simulink library "Turbine_Input_Lib"  (R2025a)
settings: Solver=ode45  StartTime=0.0  StopTime=10.0  RelTol=1e-3  EnableMultiTasking=on
undefined symbols (not defined in the file): sigbuilder_block
libraries: simulink x1, $bdroot x1
Description:
  | Copyright 2009-2025 The MathWorks, Inc. MathWorks, Inc.
settings Model: Creator=smiller  LastModifiedBy=smiller
settings SolverCC: AlgebraicLoopSolver=TrustRegion
settings DataIOCC: LimitDataPoints=on  SaveFormat=Array  SignalLoggingSaveFormat=ModelDataLogs  ReturnWorkspaceOutputs=off
settings OptimizationCC: ReuseModelBlockBuffer=off  ExpressionDepthLimit=2147483647.0  LifeSpan=inf
settings DebuggingCC: UnderspecifiedInitializationDetection=Classic  MergeDetectMultiDrivingBlocksExec=none  SolverPrmCheckMsg=warning  FcnCallInpInsideContextMsg=warning  UnconnectedInputMsg=warning  UnconnectedOutputMsg=warning  UnconnectedLineMsg=warning  AllowSymbolicDim=off  StateNameClashWarn=warning  PregeneratedLibrarySubsystemCodeDiagnostic=none  SFUnexpectedBacktrackingDiag=warning  SFNoUnconditionalDefaultTransitionDiag=warning  SFExecutionAtInitializationDiag=none  ArithmeticOperatorsInVariantConditions=warning
settings HardwareCC: ProdBitPerPointer=32.0  ProdBitPerSizeT=32.0  ProdBitPerPtrDiffT=32.0  ProdLargestAtomicFloat=None  ProdIntDivRoundTo=Undefined  ProdEndianess=Unspecified  ProdWordSize=32.0  ProdHWDeviceType=32-bit Generic
settings ModelReferenceCC: EnableRefExpFcnMdlSchedulingChecks=on  PropagateSignalLabelsOutOfModel=off
settings SFSimCC: SimUseLocalCustomCode=off  CustomCodeUndefinedFunction=UseInterfaceOnly
settings RTWCC: RTWUseLocalCustomCode=off  GPUComputeCapability=3.5  DLArmComputeVersion=19.05
settings CodeAppCC: StateflowObjectComments=on
settings GRTTargetCC: TargetLangStandard=C89/C90 (ANSI)  CombineOutputUpdateFcns=off  GRTInterface=on
settings ConfigComp: CovMetricSettings=dw  CovSaveCumulativeToWorkspaceVar=on  CovSaveSingleToWorkspaceVar=on  CovExternalEMLEnable=off  CovSFcnEnable=off

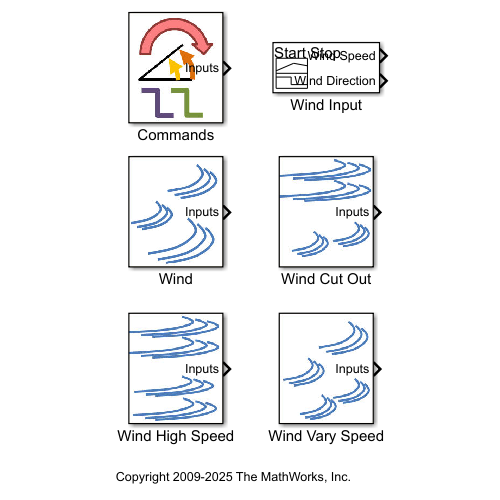
[thumbnail: Simulink's stored preview of the top-level diagram]
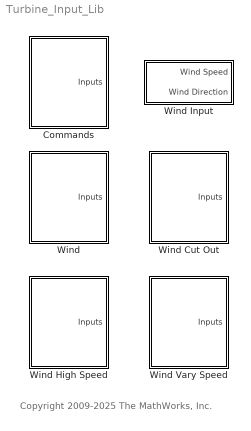
== system Turbine_Input_Lib ==
  note: Copyright 2009-2025 The MathWorks, Inc.
  Commands : Subsystem
      mask Display: image('Turbine_Input_Commands_IMAGE.jpg');
  Wind : Subsystem
      mask Display: image('Turbine_Input_Wind_IMAGE.jpg');
  Wind Cut Out : Subsystem
      mask Display: image('Turbine_Input_Wind_Cut_Out_IMAGE.jpg');
  Wind High Speed : Subsystem
      mask Display: image('Turbine_Input_Wind_High_Speed_IMAGE.jpg');
  Wind Input : Subsystem  Tag=STV Subsys  LoadFcn=sigbuilder_block('load');  StartFcn=sigbuilder_block('start');  StopFcn=sigbuilder_block('stop');  ClipboardFcn=sigbuilder_block('clipboard');  mask(Sigbuilder block){tuvar=[0:10]}
      mask help: Sigbuilder GUI
      mask init:
      | if ~strcmp(get_param(bdroot(gcbh),'SimulationStatus'),'stopped') tuvar = sigbuilder_block('maskInit'); end
      settings: CopyFcn=sigbuilder_block('copy');  DeleteFcn=sigbuilder_block('delete');  ModelCloseFcn=sigbuilder_block('modelClose');  PreSaveFcn=sigbuilder_block('preSave');  PauseFcn=sigbuilder_block('pause')  ContinueFcn=sigbuilder_block('continue')  NameChangeFcn=sigbuilder_block('namechange');  OpenFcn=sigbuilder_block('open',[-3.6 225.6 762 360.6 ]);  CloseFcn=sigbuilder_block('close');
      mask Display: plot(0, 0, 100, 100,[2, 2, 32, 32, 2], [68, 8, 8, 68, 68],[32, 2], [38, 38], [32, 19, 2],[53, 60, 44], [32, 17, 17, 2],[16, 16, 31, 31]);txt = getActiveGroup(gcbh);text(2, 100, txt,'verticalAlignment', 'top');
  Wind Vary Speed : Subsystem
      mask Display: image('Turbine_Input_Wind_Vary_Speed_IMAGE.jpg');

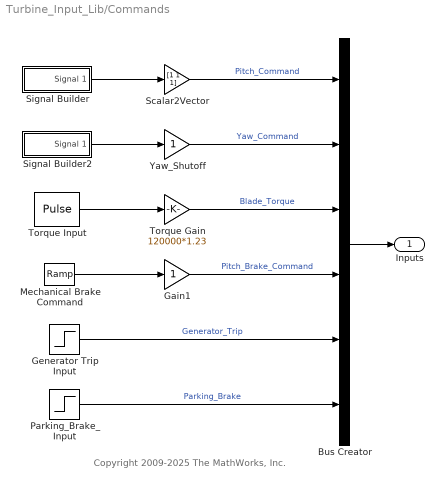
== system Turbine_Input_Lib/Commands ==
  note: Copyright 2009-2025 The MathWorks, Inc.
  Bus Creator : BusCreator  Inputs=6
  Gain1 : Gain
  Generator Trip Input : Step  Time=90  Before=1  SampleTime=0
  Mechanical Brake Command : simulink/Sources/Ramp  slope=1  start=40  InitialOutput=0
  Parking_Brake_Input : Step  Time=5  Before=1  After=0  SampleTime=0
  Scalar2Vector : Gain  Gain=[1 1 1]
  Signal Builder : Subsystem  Tag=STV Subsys  LoadFcn=sigbuilder_block('load');  StartFcn=sigbuilder_block('start');  StopFcn=sigbuilder_block('stop');  ClipboardFcn=sigbuilder_block('clipboard');  mask(Sigbuilder block){tuvar=[0:10]}
      mask help: Sigbuilder GUI
      mask init:
      | if ~strcmp(get_param(bdroot(gcbh),'SimulationStatus'),'stopped') tuvar = sigbuilder_block('maskInit'); end
      settings: CopyFcn=sigbuilder_block('copy');  DeleteFcn=sigbuilder_block('delete');  ModelCloseFcn=sigbuilder_block('modelClose');  PreSaveFcn=sigbuilder_block('preSave');  PauseFcn=sigbuilder_block('pause')  ContinueFcn=sigbuilder_block('continue')  NameChangeFcn=sigbuilder_block('namechange');  OpenFcn=sigbuilder_block('open',[214.5 254.25 550.5 399.75 ]);  CloseFcn=sigbuilder_block('close');
      mask Display: plot(0, 0, 100, 100,[2, 2, 32, 32, 2], [68, 8, 8, 68, 68],[32, 2], [38, 38], [32, 19, 2],[53, 60, 44], [32, 17, 17, 2],[16, 16, 31, 31]);txt = getActiveGroup(gcbh);text(2, 100, txt,'verticalAlignment', 'top');
  Signal Builder2 : Subsystem  Tag=STV Subsys  LoadFcn=sigbuilder_block('load');  StartFcn=sigbuilder_block('start');  StopFcn=sigbuilder_block('stop');  ClipboardFcn=sigbuilder_block('clipboard');  mask(Sigbuilder block){tuvar=[0:10]}
      mask help: Sigbuilder GUI
      mask init:
      | if ~strcmp(get_param(bdroot(gcbh),'SimulationStatus'),'stopped') tuvar = sigbuilder_block('maskInit'); end
      settings: CopyFcn=sigbuilder_block('copy');  DeleteFcn=sigbuilder_block('delete');  ModelCloseFcn=sigbuilder_block('modelClose');  PreSaveFcn=sigbuilder_block('preSave');  PauseFcn=sigbuilder_block('pause')  ContinueFcn=sigbuilder_block('continue')  NameChangeFcn=sigbuilder_block('namechange');  OpenFcn=sigbuilder_block('open',[28.5 161.25 550.5 489 ]);  CloseFcn=sigbuilder_block('close');
      mask Display: plot(0, 0, 100, 100,[2, 2, 32, 32, 2], [68, 8, 8, 68, 68],[32, 2], [38, 38], [32, 19, 2],[53, 60, 44], [32, 17, 17, 2],[16, 16, 31, 31]);txt = getActiveGroup(gcbh);text(2, 100, txt,'verticalAlignment', 'top');
  Torque Gain : Gain  Gain=120000*1.23
  Torque Input : DiscretePulseGenerator  PulseType=Time based  Amplitude=10  Period=100  PulseWidth=10
  Yaw_Shutoff : Gain
  Inputs : Outport  VectorParamsAs1DForOutWhenUnconnected=off
  wires:
  Parking_Brake_Input/1 -> Bus Creator/6  "Parking_Brake"
  Gain1/1 -> Bus Creator/4  "Pitch_Brake_Command"
  Generator Trip Input/1 -> Bus Creator/5  "Generator_Trip"
  Mechanical Brake Command/1 -> Gain1/1
  Torque Gain/1 -> Bus Creator/3  "Blade_Torque"
  Yaw_Shutoff/1 -> Bus Creator/2  "Yaw_Command"
  Scalar2Vector/1 -> Bus Creator/1  "Pitch_Command"
  Torque Input/1 -> Torque Gain/1
  Signal Builder/1(Signal 1) -> Scalar2Vector/1
  Signal Builder2/1(Signal 1) -> Yaw_Shutoff/1
  Bus Creator/1 -> Inputs/1

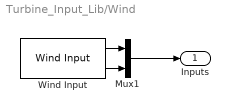
== system Turbine_Input_Lib/Wind ==
  Mux1 : Mux  Inputs=2
  Wind Input : $bdroot/Wind Input  Tag=STV Subsys  tuvar=[0:10]
  Inputs : Outport  VectorParamsAs1DForOutWhenUnconnected=off
  wires:
  Mux1/1 -> Inputs/1
  Wind Input/1 -> Mux1/1
  Wind Input/2 -> Mux1/2

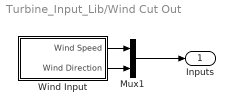
== system Turbine_Input_Lib/Wind Cut Out ==
  Mux1 : Mux  Inputs=2
  Wind Input : Subsystem  Tag=STV Subsys  AncestorBlock=Turbine_Input_Lib/Wind Input  LoadFcn=sigbuilder_block('load');  StartFcn=sigbuilder_block('start');  StopFcn=sigbuilder_block('stop');  ClipboardFcn=sigbuilder_block('clipboard');  mask(Sigbuilder block){}
      mask help: Sigbuilder GUI
      mask init:
      | if ~strcmp(get_param(bdroot(gcbh),'SimulationStatus'),'stopped') tuvar = sigbuilder_block('maskInit'); end
      settings: LibrarySourceBlock=Turbine_Input_Lib/Wind Input  CopyFcn=sigbuilder_block('copy');  DeleteFcn=sigbuilder_block('delete');  ModelCloseFcn=sigbuilder_block('modelClose');  PreSaveFcn=sigbuilder_block('preSave');  PauseFcn=sigbuilder_block('pause')  ContinueFcn=sigbuilder_block('continue')  NameChangeFcn=sigbuilder_block('namechange');  OpenFcn=sigbuilder_block('open',[-3.6 225.6 762 360.6 ]);  CloseFcn=sigbuilder_block('close');
      mask Display: plot(0, 0, 100, 100,[2, 2, 32, 32, 2], [68, 8, 8, 68, 68],[32, 2], [38, 38], [32, 19, 2],[53, 60, 44], [32, 17, 17, 2],[16, 16, 31, 31]);txt = getActiveGroup(gcbh);text(2, 100, txt,'verticalAlignment', 'top');
  Inputs : Outport  VectorParamsAs1DForOutWhenUnconnected=off
  wires:
  Mux1/1 -> Inputs/1
  Wind Input/1(Wind Speed) -> Mux1/1
  Wind Input/2(Wind Direction) -> Mux1/2

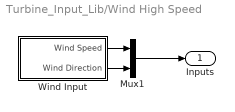
== system Turbine_Input_Lib/Wind High Speed ==
  Mux1 : Mux  Inputs=2
  Wind Input : Subsystem  Tag=STV Subsys  AncestorBlock=Turbine_Input_Lib/Wind Input  LoadFcn=sigbuilder_block('load');  StartFcn=sigbuilder_block('start');  StopFcn=sigbuilder_block('stop');  ClipboardFcn=sigbuilder_block('clipboard');  mask(Sigbuilder block){}
      mask help: Sigbuilder GUI
      mask init:
      | if ~strcmp(get_param(bdroot(gcbh),'SimulationStatus'),'stopped') tuvar = sigbuilder_block('maskInit'); end
      settings: LibrarySourceBlock=Turbine_Input_Lib/Wind Input  CopyFcn=sigbuilder_block('copy');  DeleteFcn=sigbuilder_block('delete');  ModelCloseFcn=sigbuilder_block('modelClose');  PreSaveFcn=sigbuilder_block('preSave');  PauseFcn=sigbuilder_block('pause')  ContinueFcn=sigbuilder_block('continue')  NameChangeFcn=sigbuilder_block('namechange');  OpenFcn=sigbuilder_block('open',[-3.6 225.6 762 360.6 ]);  CloseFcn=sigbuilder_block('close');
      mask Display: plot(0, 0, 100, 100,[2, 2, 32, 32, 2], [68, 8, 8, 68, 68],[32, 2], [38, 38], [32, 19, 2],[53, 60, 44], [32, 17, 17, 2],[16, 16, 31, 31]);txt = getActiveGroup(gcbh);text(2, 100, txt,'verticalAlignment', 'top');
  Inputs : Outport  VectorParamsAs1DForOutWhenUnconnected=off
  wires:
  Wind Input/2(Wind Direction) -> Mux1/2
  Wind Input/1(Wind Speed) -> Mux1/1
  Mux1/1 -> Inputs/1

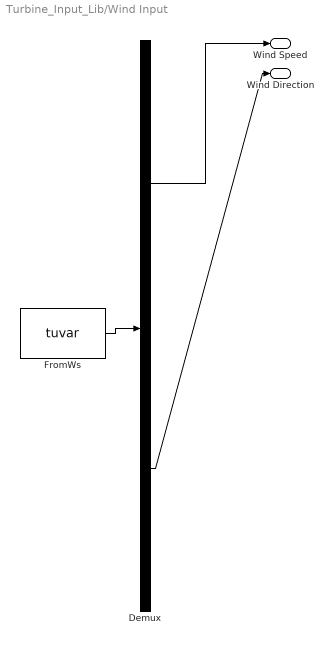
== system Turbine_Input_Lib/Wind Input ==
  Demux : Demux  Tag=STV Demux  Outputs=2
      settings: DisplayOption=none
  FromWs : FromWorkspace  Tag=STV FromWs  VariableName=tuvar
      SigBuilderData=|
      | common.afterFinalStr = 'Extrapolate'
      | common.sampleTime = 0
      | dataSet(1).timeRange = [0 130]
      | dataSet(1).name = 'Constant Wind No Yaw'
      | dataSet(2).timeRange = [0 130]
      | dataSet(2).name = 'Constant Wind'
      | dataSet(3).timeRange = [0 130]
      | dataSet(3).name = 'High WS No Yaw'
      | dataSet(4).timeRange = [0 60]
      | dataSet(4).name = 'High Wind Speed'
      | dataSet(5).timeRange = [0 130]
      | dataSet(5).name = 'Cut Out'
      | dataSet(6).timeRange = [0 130]
      | dataSet(6).name = 'Start Stop'
      | dataSet(7).timeRange = [0 130]
      | dataSet(7).name = 'Start Stop No Yaw'
      | sbobj.Groups(1).Name = 'Constant Wind No Yaw'
      | sbobj.Groups(1).Signals(1).Name = 'Wind Speed'
      | sbobj.Groups(1).Signals(1).XData = [0 10 130]
      | sbobj.Groups(1).Signals(1).YData = [10 10 10]
      | sbobj.Groups(1).Signals(2).Name = 'Wind Direction'
      | sbobj.Groups(1).Signals(2).XData = [0 1 11 21 31 130]
      | sbobj.Groups(1).Signals(2).YData = [0 0 0 0 0 0]
      | sbobj.Groups(1).TimeRange = [0 130]
      | sbobj.Groups(2).Name = 'Constant Wind'
      | sbobj.Groups(2).Signals(1).Name = 'Wind Speed'
      | sbobj.Groups(2).Signals(1).XData = [0 10 130]
      | sbobj.Groups(2).Signals(1).YData = [10 10 10]
      | sbobj.Groups(2).Signals(2).Name = 'Wind Direction'
      | sbobj.Groups(2).Signals(2).XData = [0 1 1 11 11 21 21 31 31 130]
      | sbobj.Groups(2).Signals(2).YData = [0 0 4 4 0 0 -4 -4 0 0]
      | sbobj.Groups(2).TimeRange = [0 130]
      | sbobj.Groups(3).Name = 'High WS No Yaw'
      | sbobj.Groups(3).Signals(1).Name = 'Wind Speed'
      | sbobj.Groups(3).Signals(1).XData = [0 10 10 25.1 28 91.8 100 130]
      | sbobj.Groups(3).Signals(1).YData = [10 10 9.9 9.9 5 5 8 10]
      | sbobj.Groups(3).Signals(2).Name = 'Wind Direction'
      | sbobj.Groups(3).Signals(2).XData = [0 1 11 21 21 31 31 130]
      | sbobj.Groups(3).Signals(2).YData = [0 0 0 0 0 0 0 0]
      | sbobj.Groups(3).TimeRange = [0 130]
      | sbobj.Groups(4).Name = 'High Wind Speed'
      | sbobj.Groups(4).Signals(1).Name = 'Wind Speed'
      | sbobj.Groups(4).Signals(1).XData = [0 10 60]
      | sbobj.Groups(4).Signals(1).YData = [10 9.9 25]
      | sbobj.Groups(4).Signals(2).Name = 'Wind Direction'
      | sbobj.Groups(4).Signals(2).XData = [0 1 11 21 31 60]
      | sbobj.Groups(4).Signals(2).YData = [0 0 4 0 -2.1 0]
      | sbobj.Groups(4).TimeRange = [0 60]
      | sbobj.Groups(5).Name = 'Cut Out'
      | sbobj.Groups(5).Signals(1).Name = 'Wind Speed'
      | sbobj.Groups(5).Signals(1).XData = [0 5 25.1 28 60 75 121.8 130]
      | sbobj.Groups(5).Signals(1).YData = [10 10 8.7 7.85 9.65 2 2 2]
      | sbobj.Groups(5).Signals(2).Name = 'Wind Direction'
      | sbobj.Groups(5).Signals(2).XData = [0 1 1 11 11 21 21 31 31 130]
      | sbobj.Groups(5).Signals(2).YData = [0 0 4 4 0 0 -4 -4 0 0]
      | sbobj.Groups(5).TimeRange = [0 130]
      | sbobj.Groups(6).Name = 'Start Stop'
      | sbobj.Groups(6).Signals(1).Name = 'Wind Speed'
      | sbobj.Groups(6).Signals(1).XData = [0 5 25 28 55 75 80 130]
      | sbobj.Groups(6).Signals(1).YData = [2 2 13 10 15 2 2 2]
      | sbobj.Groups(6).Signals(2).Name = 'Wind Direction'
      | sbobj.Groups(6).Signals(2).XData = [0 1 11 21 31 36.6 54.8 75 130]
      | sbobj.Groups(6).Signals(2).YData = [0 0 2.9 0.5 0.5 1.57171717172 -4 -4 -4]
      | sbobj.Groups(6).TimeRange = [0 130]
      | sbobj.Groups(7).Name = 'Start Stop No Yaw'
      | sbobj.Groups(7).Signals(1).Name = 'Wind Speed'
      | sbobj.Groups(7).Signals(1).XData = [0 5 25 28 55 75 80 130]
      | sbobj.Groups(7).Signals(1).YData = [2 2 13 10 15 2 2 2]
      | sbobj.Groups(7).Signals(2).Name = 'Wind Direction'
      | sbobj.Groups(7).Signals(2).XData = [0 130]
      | sbobj.Groups(7).Signals(2).YData = [0 0]
      | sbobj.Groups(7).TimeRange = [0 130]
  Wind Speed : Outport  Tag=STV Outport  VectorParamsAs1DForOutWhenUnconnected=off
  Wind Direction : Outport  Tag=STV Outport  Port=2  VectorParamsAs1DForOutWhenUnconnected=off
  wires:
  Demux/2 -> Wind Direction/1
  Demux/1 -> Wind Speed/1
  FromWs/1 -> Demux/1

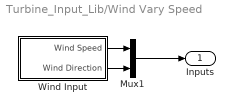
== system Turbine_Input_Lib/Wind Vary Speed ==
  Mux1 : Mux  Inputs=2
  Wind Input : Subsystem  Tag=STV Subsys  AncestorBlock=Turbine_Input_Lib/Wind Input  LoadFcn=sigbuilder_block('load');  StartFcn=sigbuilder_block('start');  StopFcn=sigbuilder_block('stop');  ClipboardFcn=sigbuilder_block('clipboard');  mask(Sigbuilder block){}
      mask help: Sigbuilder GUI
      mask init:
      | if ~strcmp(get_param(bdroot(gcbh),'SimulationStatus'),'stopped') tuvar = sigbuilder_block('maskInit'); end
      settings: LibrarySourceBlock=Turbine_Input_Lib/Wind Input  CopyFcn=sigbuilder_block('copy');  DeleteFcn=sigbuilder_block('delete');  ModelCloseFcn=sigbuilder_block('modelClose');  PreSaveFcn=sigbuilder_block('preSave');  PauseFcn=sigbuilder_block('pause')  ContinueFcn=sigbuilder_block('continue')  NameChangeFcn=sigbuilder_block('namechange');  OpenFcn=sigbuilder_block('open',[-3.6 225.6 762 360.6 ]);  CloseFcn=sigbuilder_block('close');
      mask Display: plot(0, 0, 100, 100,[2, 2, 32, 32, 2], [68, 8, 8, 68, 68],[32, 2], [38, 38], [32, 19, 2],[53, 60, 44], [32, 17, 17, 2],[16, 16, 31, 31]);txt = getActiveGroup(gcbh);text(2, 100, txt,'verticalAlignment', 'top');
  Inputs : Outport  VectorParamsAs1DForOutWhenUnconnected=off
  wires:
  Wind Input/2(Wind Direction) -> Mux1/2
  Wind Input/1(Wind Speed) -> Mux1/1
  Mux1/1 -> Inputs/1

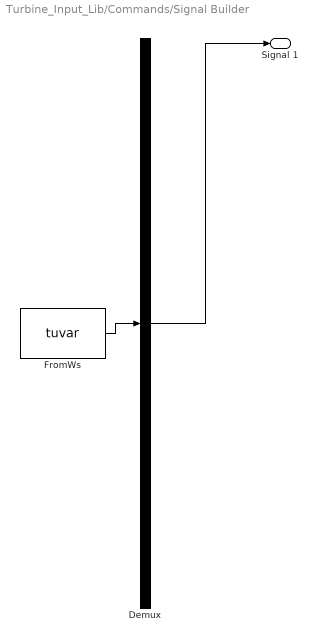
== system Turbine_Input_Lib/Commands/Signal Builder ==
  Demux : Demux  Tag=STV Demux  Outputs=1
      settings: DisplayOption=none
  FromWs : FromWorkspace  Tag=STV FromWs  VariableName=tuvar
      SigBuilderData=|
      | common.afterFinalStr = 'Extrapolate'
      | common.sampleTime = 0
      | dataSet(1).timeRange = [0 50]
      | dataSet(1).name = 'Pos_Test'
      | dataSet(2).timeRange = [0 50]
      | dataSet(2).name = 'Pos_Neg_Test'
      | dataSet(3).timeRange = [0 50]
      | dataSet(3).name = 'Step_Test'
      | sbobj.Groups(1).Name = 'Pos_Test'
      | sbobj.Groups(1).Signals.Name = 'Signal 1'
      | sbobj.Groups(1).Signals.XData = [0 5 5 7.5 7.5 25.1 25.1 28 28 50]
      | sbobj.Groups(1).Signals.YData = [0 0 20 20 0 0 20 20 0 0]
      | sbobj.Groups(1).TimeRange = [0 50]
      | sbobj.Groups(2).Name = 'Pos_Neg_Test'
      | sbobj.Groups(2).Signals.Name = 'Signal 1'
      | sbobj.Groups(2).Signals.XData = [0 3 3 5.5 5.5 8 8 10.5 10.5 50]
      | sbobj.Groups(2).Signals.YData = [0 0 20 20 0 0 -20 -20 0 0]
      | sbobj.Groups(2).TimeRange = [0 50]
      | sbobj.Groups(3).Name = 'Step_Test'
      | sbobj.Groups(3).Signals.Name = 'Signal 1'
      | sbobj.Groups(3).Signals.XData = [0 1 1 7.5 25.1 30 30 50]
      | sbobj.Groups(3).Signals.YData = [0 0 20 20 20 20 0 0]
      | sbobj.Groups(3).TimeRange = [0 50]
  Signal 1 : Outport  Tag=STV Outport  VectorParamsAs1DForOutWhenUnconnected=off
  wires:
  FromWs/1 -> Demux/1
  Demux/1 -> Signal 1/1

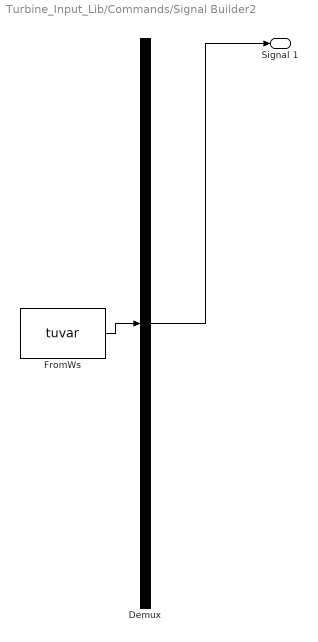
== system Turbine_Input_Lib/Commands/Signal Builder2 ==
  Demux : Demux  Tag=STV Demux  Outputs=1
      settings: DisplayOption=none
  FromWs : FromWorkspace  Tag=STV FromWs  VariableName=tuvar
      SigBuilderData=|
      | common.afterFinalStr = 'Extrapolate'
      | common.sampleTime = 0
      | dataSet(1).timeRange = [0 50]
      | dataSet(1).name = 'Pos_Neg_Test'
      | dataSet(2).timeRange = [0 50]
      | dataSet(2).name = 'Step_Test'
      | dataSet(3).timeRange = [0 50]
      | dataSet(3).name = 'Ramp_Test'
      | sbobj.Groups(1).Name = 'Pos_Neg_Test'
      | sbobj.Groups(1).Signals.Name = 'Signal 1'
      | sbobj.Groups(1).Signals.XData = [0 1 1 11 11 21 21 31 31 50]
      | sbobj.Groups(1).Signals.YData = [0 0 4 4 0 0 -4 -4 0 0]
      | sbobj.Groups(2).Name = 'Step_Test'
      | sbobj.Groups(2).Signals.Name = 'Signal 1'
      | sbobj.Groups(2).Signals.XData = [0 1 1 11 21 31 31 50]
      | sbobj.Groups(2).Signals.YData = [0 0 4 4 4 4 0 0]
      | sbobj.Groups(3).Name = 'Ramp_Test'
      | sbobj.Groups(3).Signals.Name = 'Signal 1'
      | sbobj.Groups(3).Signals.XData = [0 1 1 11 21 31 39.1 50]
      | sbobj.Groups(3).Signals.YData = [0 0 2.46 4 2.32 3.18 1.16 0]
  Signal 1 : Outport  Tag=STV Outport  VectorParamsAs1DForOutWhenUnconnected=off
  wires:
  FromWs/1 -> Demux/1
  Demux/1 -> Signal 1/1

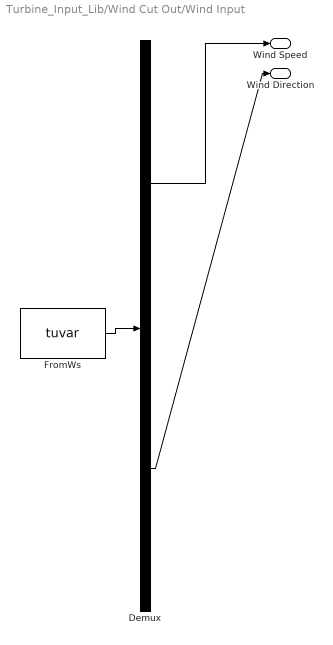
== system Turbine_Input_Lib/Wind Cut Out/Wind Input ==
  Demux : Demux  Tag=STV Demux  Outputs=2
      settings: DisplayOption=none
  FromWs : FromWorkspace  Tag=STV FromWs  VariableName=tuvar
      SigBuilderData=|
      | common.afterFinalStr = 'Extrapolate'
      | common.sampleTime = 0
      | dataSet(1).timeRange = [0 130]
      | dataSet(1).name = 'Constant Wind No Yaw'
      | dataSet(2).timeRange = [0 130]
      | dataSet(2).name = 'Constant Wind'
      | dataSet(3).timeRange = [0 60]
      | dataSet(3).name = 'High Wind Speed'
      | dataSet(4).timeRange = [0 130]
      | dataSet(4).name = 'Cut Out'
      | dataSet(5).timeRange = [0 130]
      | dataSet(5).name = 'Start Stop'
      | dataSet(6).timeRange = [0 130]
      | dataSet(6).name = 'Start Stop No Yaw'
      | dataSet(7).timeRange = [0 130]
      | dataSet(7).name = 'Varying Wind'
      | sbobj.Groups(1).Name = 'Constant Wind No Yaw'
      | sbobj.Groups(1).Signals(1).Name = 'Wind Speed'
      | sbobj.Groups(1).Signals(1).XData = [0 10 130]
      | sbobj.Groups(1).Signals(1).YData = [10 10 10]
      | sbobj.Groups(1).Signals(2).Name = 'Wind Direction'
      | sbobj.Groups(1).Signals(2).XData = [0 1 11 21 31 130]
      | sbobj.Groups(1).Signals(2).YData = [0 0 0 0 0 0]
      | sbobj.Groups(1).TimeRange = [0 130]
      | sbobj.Groups(2).Name = 'Constant Wind'
      | sbobj.Groups(2).Signals(1).Name = 'Wind Speed'
      | sbobj.Groups(2).Signals(1).XData = [0 10 130]
      | sbobj.Groups(2).Signals(1).YData = [10 10 10]
      | sbobj.Groups(2).Signals(2).Name = 'Wind Direction'
      | sbobj.Groups(2).Signals(2).XData = [0 1 1 11 11 21 21 31 31 130]
      | sbobj.Groups(2).Signals(2).YData = [0 0 4 4 0 0 -4 -4 0 0]
      | sbobj.Groups(2).TimeRange = [0 130]
      | sbobj.Groups(3).Name = 'High Wind Speed'
      | sbobj.Groups(3).Signals(1).Name = 'Wind Speed'
      | sbobj.Groups(3).Signals(1).XData = [0 10 60]
      | sbobj.Groups(3).Signals(1).YData = [10 9.9 25]
      | sbobj.Groups(3).Signals(2).Name = 'Wind Direction'
      | sbobj.Groups(3).Signals(2).XData = [0 1 11 21 31 60]
      | sbobj.Groups(3).Signals(2).YData = [0 0 4 0 -2.1 0]
      | sbobj.Groups(3).TimeRange = [0 60]
      | sbobj.Groups(4).Name = 'Cut Out'
      | sbobj.Groups(4).Signals(1).Name = 'Wind Speed'
      | sbobj.Groups(4).Signals(1).XData = [0 5 25.1 28 60 75 121.8 130]
      | sbobj.Groups(4).Signals(1).YData = [10 10 8.7 7.85 9.65 2 2 2]
      | sbobj.Groups(4).Signals(2).Name = 'Wind Direction'
      | sbobj.Groups(4).Signals(2).XData = [0 1 1 11 11 21 21 31 31 130]
      | sbobj.Groups(4).Signals(2).YData = [0 0 4 4 0 0 -4 -4 0 0]
      | sbobj.Groups(4).TimeRange = [0 130]
      | sbobj.Groups(5).Name = 'Start Stop'
      | sbobj.Groups(5).Signals(1).Name = 'Wind Speed'
      | sbobj.Groups(5).Signals(1).XData = [0 5 25 28 55 75 80 130]
      | sbobj.Groups(5).Signals(1).YData = [2 2 13 10 15 2 2 2]
      | sbobj.Groups(5).Signals(2).Name = 'Wind Direction'
      | sbobj.Groups(5).Signals(2).XData = [0 1 11 21 31 36.6 54.8 75 130]
      | sbobj.Groups(5).Signals(2).YData = [0 0 2.9 0.5 0.5 1.57171717172 -4 -4 -4]
      | sbobj.Groups(5).TimeRange = [0 130]
      | sbobj.Groups(6).Name = 'Start Stop No Yaw'
      | sbobj.Groups(6).Signals(1).Name = 'Wind Speed'
      | sbobj.Groups(6).Signals(1).XData = [0 5 25 28 55 75 80 130]
      | sbobj.Groups(6).Signals(1).YData = [2 2 13 10 15 2 2 2]
      | sbobj.Groups(6).Signals(2).Name = 'Wind Direction'
      | sbobj.Groups(6).Signals(2).XData = [0 130]
      | sbobj.Groups(6).Signals(2).YData = [0 0]
      | sbobj.Groups(6).TimeRange = [0 130]
      | sbobj.Groups(7).Name = 'Varying Wind'
      | sbobj.Groups(7).Signals(1).Name = 'Wind Speed'
      | sbobj.Groups(7).Signals(1).XData = [0 5 25 28 45 60.2 75 78.2 80 130]
      | sbobj.Groups(7).Signals(1).YData = [2 2 13 10 14.4 10.6 13.9 8 8 2]
      | sbobj.Groups(7).Signals(2).Name = 'Wind Direction'
      | sbobj.Groups(7).Signals(2).XData = [0 1 11 21 31 36.6 54.8 75 130]
      | sbobj.Groups(7).Signals(2).YData = [0 0 2.9 0.5 0.5 1.57171717172 -4 -4 -4]
      | sbobj.Groups(7).TimeRange = [0 130]
  Wind Speed : Outport  Tag=STV Outport  VectorParamsAs1DForOutWhenUnconnected=off
  Wind Direction : Outport  Tag=STV Outport  Port=2  VectorParamsAs1DForOutWhenUnconnected=off
  wires:
  Demux/2 -> Wind Direction/1
  Demux/1 -> Wind Speed/1
  FromWs/1 -> Demux/1

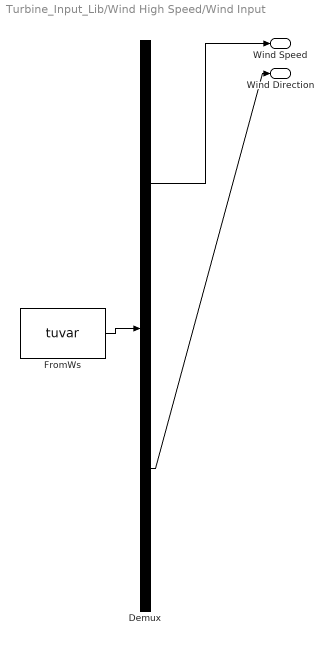
== system Turbine_Input_Lib/Wind High Speed/Wind Input ==
  Demux : Demux  Tag=STV Demux  Outputs=2
      settings: DisplayOption=none
  FromWs : FromWorkspace  Tag=STV FromWs  VariableName=tuvar
      SigBuilderData=|
      | common.afterFinalStr = 'Extrapolate'
      | common.sampleTime = 0
      | dataSet(1).timeRange = [0 130]
      | dataSet(1).name = 'Constant Wind No Yaw'
      | dataSet(2).timeRange = [0 130]
      | dataSet(2).name = 'Constant Wind'
      | dataSet(3).timeRange = [0 60]
      | dataSet(3).name = 'High Wind Speed'
      | dataSet(4).timeRange = [0 130]
      | dataSet(4).name = 'Cut Out'
      | dataSet(5).timeRange = [0 130]
      | dataSet(5).name = 'Start Stop'
      | dataSet(6).timeRange = [0 130]
      | dataSet(6).name = 'Start Stop No Yaw'
      | dataSet(7).timeRange = [0 130]
      | dataSet(7).name = 'Varying Wind'
      | sbobj.Groups(1).Name = 'Constant Wind No Yaw'
      | sbobj.Groups(1).Signals(1).Name = 'Wind Speed'
      | sbobj.Groups(1).Signals(1).XData = [0 10 130]
      | sbobj.Groups(1).Signals(1).YData = [10 10 10]
      | sbobj.Groups(1).Signals(2).Name = 'Wind Direction'
      | sbobj.Groups(1).Signals(2).XData = [0 1 11 21 31 130]
      | sbobj.Groups(1).Signals(2).YData = [0 0 0 0 0 0]
      | sbobj.Groups(1).TimeRange = [0 130]
      | sbobj.Groups(2).Name = 'Constant Wind'
      | sbobj.Groups(2).Signals(1).Name = 'Wind Speed'
      | sbobj.Groups(2).Signals(1).XData = [0 10 130]
      | sbobj.Groups(2).Signals(1).YData = [10 10 10]
      | sbobj.Groups(2).Signals(2).Name = 'Wind Direction'
      | sbobj.Groups(2).Signals(2).XData = [0 1 1 11 11 21 21 31 31 130]
      | sbobj.Groups(2).Signals(2).YData = [0 0 4 4 0 0 -4 -4 0 0]
      | sbobj.Groups(2).TimeRange = [0 130]
      | sbobj.Groups(3).Name = 'High Wind Speed'
      | sbobj.Groups(3).Signals(1).Name = 'Wind Speed'
      | sbobj.Groups(3).Signals(1).XData = [0 10 60]
      | sbobj.Groups(3).Signals(1).YData = [10 9.9 25]
      | sbobj.Groups(3).Signals(2).Name = 'Wind Direction'
      | sbobj.Groups(3).Signals(2).XData = [0 1 11 21 31 60]
      | sbobj.Groups(3).Signals(2).YData = [0 0 4 0 -2.1 0]
      | sbobj.Groups(3).TimeRange = [0 60]
      | sbobj.Groups(4).Name = 'Cut Out'
      | sbobj.Groups(4).Signals(1).Name = 'Wind Speed'
      | sbobj.Groups(4).Signals(1).XData = [0 5 25.1 28 60 75 121.8 130]
      | sbobj.Groups(4).Signals(1).YData = [10 10 8.7 7.85 9.65 2 2 2]
      | sbobj.Groups(4).Signals(2).Name = 'Wind Direction'
      | sbobj.Groups(4).Signals(2).XData = [0 1 1 11 11 21 21 31 31 130]
      | sbobj.Groups(4).Signals(2).YData = [0 0 4 4 0 0 -4 -4 0 0]
      | sbobj.Groups(4).TimeRange = [0 130]
      | sbobj.Groups(5).Name = 'Start Stop'
      | sbobj.Groups(5).Signals(1).Name = 'Wind Speed'
      | sbobj.Groups(5).Signals(1).XData = [0 5 25 28 55 75 80 130]
      | sbobj.Groups(5).Signals(1).YData = [2 2 13 10 15 2 2 2]
      | sbobj.Groups(5).Signals(2).Name = 'Wind Direction'
      | sbobj.Groups(5).Signals(2).XData = [0 1 11 21 31 36.6 54.8 75 130]
      | sbobj.Groups(5).Signals(2).YData = [0 0 2.9 0.5 0.5 1.57171717172 -4 -4 -4]
      | sbobj.Groups(5).TimeRange = [0 130]
      | sbobj.Groups(6).Name = 'Start Stop No Yaw'
      | sbobj.Groups(6).Signals(1).Name = 'Wind Speed'
      | sbobj.Groups(6).Signals(1).XData = [0 5 25 28 55 75 80 130]
      | sbobj.Groups(6).Signals(1).YData = [2 2 13 10 15 2 2 2]
      | sbobj.Groups(6).Signals(2).Name = 'Wind Direction'
      | sbobj.Groups(6).Signals(2).XData = [0 130]
      | sbobj.Groups(6).Signals(2).YData = [0 0]
      | sbobj.Groups(6).TimeRange = [0 130]
      | sbobj.Groups(7).Name = 'Varying Wind'
      | sbobj.Groups(7).Signals(1).Name = 'Wind Speed'
      | sbobj.Groups(7).Signals(1).XData = [0 5 25 28 45 60.2 75 78.2 80 130]
      | sbobj.Groups(7).Signals(1).YData = [2 2 13 10 14.4 10.6 13.9 8 8 2]
      | sbobj.Groups(7).Signals(2).Name = 'Wind Direction'
      | sbobj.Groups(7).Signals(2).XData = [0 1 11 21 31 36.6 54.8 75 130]
      | sbobj.Groups(7).Signals(2).YData = [0 0 2.9 0.5 0.5 1.57171717172 -4 -4 -4]
      | sbobj.Groups(7).TimeRange = [0 130]
  Wind Speed : Outport  Tag=STV Outport  VectorParamsAs1DForOutWhenUnconnected=off
  Wind Direction : Outport  Tag=STV Outport  Port=2  VectorParamsAs1DForOutWhenUnconnected=off
  wires:
  FromWs/1 -> Demux/1
  Demux/1 -> Wind Speed/1
  Demux/2 -> Wind Direction/1

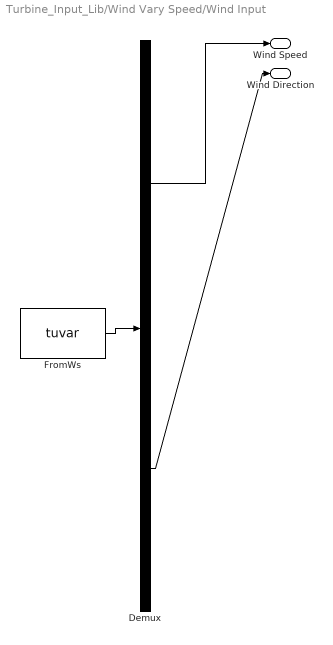
== system Turbine_Input_Lib/Wind Vary Speed/Wind Input ==
  Demux : Demux  Tag=STV Demux  Outputs=2
      settings: DisplayOption=none
  FromWs : FromWorkspace  Tag=STV FromWs  VariableName=tuvar
      SigBuilderData=|
      | common.afterFinalStr = 'Extrapolate'
      | common.sampleTime = 0
      | dataSet(1).timeRange = [0 130]
      | dataSet(1).name = 'Constant Wind No Yaw'
      | dataSet(2).timeRange = [0 130]
      | dataSet(2).name = 'Constant Wind'
      | dataSet(3).timeRange = [0 60]
      | dataSet(3).name = 'High Wind Speed'
      | dataSet(4).timeRange = [0 130]
      | dataSet(4).name = 'Cut Out'
      | dataSet(5).timeRange = [0 130]
      | dataSet(5).name = 'Start Stop'
      | dataSet(6).timeRange = [0 130]
      | dataSet(6).name = 'Start Stop No Yaw'
      | dataSet(7).timeRange = [0 130]
      | dataSet(7).name = 'Varying Wind'
      | sbobj.Groups(1).Name = 'Constant Wind No Yaw'
      | sbobj.Groups(1).Signals(1).Name = 'Wind Speed'
      | sbobj.Groups(1).Signals(1).XData = [0 10 130]
      | sbobj.Groups(1).Signals(1).YData = [10 10 10]
      | sbobj.Groups(1).Signals(2).Name = 'Wind Direction'
      | sbobj.Groups(1).Signals(2).XData = [0 1 11 21 31 130]
      | sbobj.Groups(1).Signals(2).YData = [0 0 0 0 0 0]
      | sbobj.Groups(1).TimeRange = [0 130]
      | sbobj.Groups(2).Name = 'Constant Wind'
      | sbobj.Groups(2).Signals(1).Name = 'Wind Speed'
      | sbobj.Groups(2).Signals(1).XData = [0 10 130]
      | sbobj.Groups(2).Signals(1).YData = [10 10 10]
      | sbobj.Groups(2).Signals(2).Name = 'Wind Direction'
      | sbobj.Groups(2).Signals(2).XData = [0 1 1 11 11 21 21 31 31 130]
      | sbobj.Groups(2).Signals(2).YData = [0 0 4 4 0 0 -4 -4 0 0]
      | sbobj.Groups(2).TimeRange = [0 130]
      | sbobj.Groups(3).Name = 'High Wind Speed'
      | sbobj.Groups(3).Signals(1).Name = 'Wind Speed'
      | sbobj.Groups(3).Signals(1).XData = [0 10 60]
      | sbobj.Groups(3).Signals(1).YData = [10 9.9 25]
      | sbobj.Groups(3).Signals(2).Name = 'Wind Direction'
      | sbobj.Groups(3).Signals(2).XData = [0 1 11 21 31 60]
      | sbobj.Groups(3).Signals(2).YData = [0 0 4 0 -2.1 0]
      | sbobj.Groups(3).TimeRange = [0 60]
      | sbobj.Groups(4).Name = 'Cut Out'
      | sbobj.Groups(4).Signals(1).Name = 'Wind Speed'
      | sbobj.Groups(4).Signals(1).XData = [0 5 25.1 28 60 75 121.8 130]
      | sbobj.Groups(4).Signals(1).YData = [10 10 8.7 7.85 9.65 2 2 2]
      | sbobj.Groups(4).Signals(2).Name = 'Wind Direction'
      | sbobj.Groups(4).Signals(2).XData = [0 1 1 11 11 21 21 31 31 130]
      | sbobj.Groups(4).Signals(2).YData = [0 0 4 4 0 0 -4 -4 0 0]
      | sbobj.Groups(4).TimeRange = [0 130]
      | sbobj.Groups(5).Name = 'Start Stop'
      | sbobj.Groups(5).Signals(1).Name = 'Wind Speed'
      | sbobj.Groups(5).Signals(1).XData = [0 5 25 28 55 75 80 130]
      | sbobj.Groups(5).Signals(1).YData = [2 2 13 10 15 2 2 2]
      | sbobj.Groups(5).Signals(2).Name = 'Wind Direction'
      | sbobj.Groups(5).Signals(2).XData = [0 1 11 21 31 36.6 54.8 75 130]
      | sbobj.Groups(5).Signals(2).YData = [0 0 2.9 0.5 0.5 1.57171717172 -4 -4 -4]
      | sbobj.Groups(5).TimeRange = [0 130]
      | sbobj.Groups(6).Name = 'Start Stop No Yaw'
      | sbobj.Groups(6).Signals(1).Name = 'Wind Speed'
      | sbobj.Groups(6).Signals(1).XData = [0 5 25 28 55 75 80 130]
      | sbobj.Groups(6).Signals(1).YData = [2 2 13 10 15 2 2 2]
      | sbobj.Groups(6).Signals(2).Name = 'Wind Direction'
      | sbobj.Groups(6).Signals(2).XData = [0 130]
      | sbobj.Groups(6).Signals(2).YData = [0 0]
      | sbobj.Groups(6).TimeRange = [0 130]
      | sbobj.Groups(7).Name = 'Varying Wind'
      | sbobj.Groups(7).Signals(1).Name = 'Wind Speed'
      | sbobj.Groups(7).Signals(1).XData = [0 5 25 28 45 60.2 75 78.2 80 130]
      | sbobj.Groups(7).Signals(1).YData = [2 2 13 10 14.4 10.6 13.9 8 8 2]
      | sbobj.Groups(7).Signals(2).Name = 'Wind Direction'
      | sbobj.Groups(7).Signals(2).XData = [0 1 11 21 31 36.6 54.8 75 130]
      | sbobj.Groups(7).Signals(2).YData = [0 0 2.9 0.5 0.5 1.57171717172 -4 -4 -4]
      | sbobj.Groups(7).TimeRange = [0 130]
  Wind Speed : Outport  Tag=STV Outport  VectorParamsAs1DForOutWhenUnconnected=off
  Wind Direction : Outport  Tag=STV Outport  Port=2  VectorParamsAs1DForOutWhenUnconnected=off
  wires:
  FromWs/1 -> Demux/1
  Demux/1 -> Wind Speed/1
  Demux/2 -> Wind Direction/1
